simulink model "ieee14_fault"  (R2025b)
settings: Solver=ode23t  StartTime=0.0  StopTime=0.12  FixedStep=0.2  RelTol=1e-4  AbsTol=1e-6  EnableMultiTasking=on
undefined symbols (not defined in the file or in its folder): D1, Delta
libraries: spsDiodeLib x84, spsGroundLib x84, spsSeriesRLCBranchLib x84, spsDCVoltageSourceLib x84, spsBreakerLib x42, spsThreePhaseSeriesRLCBranchLib x20, spsThreePhaseVIMeasurementLib x16, spsThreePhaseFaultLib x14, spsThreePhaseSeriesRLCLoadLib x11, spsThreePhaseSourceLib x5, spsThreePhaseTransformerTwoWindingsLib x5, spspowerguiLib x1
(part 2 of 3)

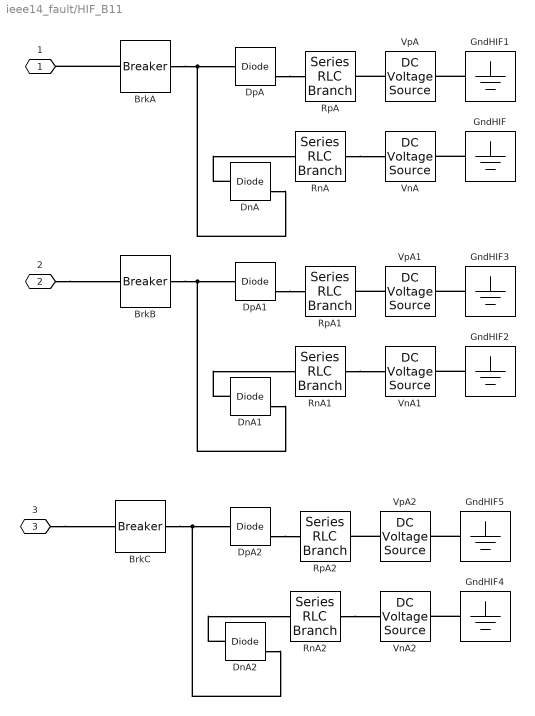
== system ieee14_fault/HIF_B11 ==
  BrkA : spsBreakerLib/Breaker  InitialState=0  SwitchingTimes=[100]  External=off  BreakerResistance=0.01  SnubberResistance=1e6  SnubberCapacitance=inf  Measurements=None  MoreParameters=on  NoBreakLoop=off
  BrkB : spsBreakerLib/Breaker  InitialState=0  SwitchingTimes=[100]  External=off  BreakerResistance=0.01  SnubberResistance=1e6  SnubberCapacitance=inf  Measurements=None  MoreParameters=on  NoBreakLoop=off
  BrkC : spsBreakerLib/Breaker  InitialState=0  SwitchingTimes=[100]  External=off  BreakerResistance=0.01  SnubberResistance=1e6  SnubberCapacitance=inf  Measurements=None  MoreParameters=on  NoBreakLoop=off
  DnA : spsDiodeLib/Diode  Ron=0.001  Lon=0  Vf=0.8  IC=0  UseSnubber=0  Rs=1e6  Cs=inf  Measurements=on
  DnA1 : spsDiodeLib/Diode  Ron=0.001  Lon=0  Vf=0.8  IC=0  UseSnubber=0  Rs=1e6  Cs=inf  Measurements=on
  DnA2 : spsDiodeLib/Diode  Ron=0.001  Lon=0  Vf=0.8  IC=0  UseSnubber=0  Rs=1e6  Cs=inf  Measurements=on
  DpA : spsDiodeLib/Diode  Ron=0.001  Lon=0  Vf=0.8  IC=0  UseSnubber=0  Rs=1e6  Cs=inf  Measurements=on
  DpA1 : spsDiodeLib/Diode  Ron=0.001  Lon=0  Vf=0.8  IC=0  UseSnubber=0  Rs=1e6  Cs=inf  Measurements=on
  DpA2 : spsDiodeLib/Diode  Ron=0.001  Lon=0  Vf=0.8  IC=0  UseSnubber=0  Rs=1e6  Cs=inf  Measurements=on
  GndHIF{,1..5} (6 alike) : spsGroundLib/Ground  LConnTagsString=a
  RnA : spsSeriesRLCBranchLib/Series RLC Branch  LConnTagsString=__new0  RConnTagsString=__new0  BranchType=R  Resistance=160  Inductance=1e-3  SetiL0=off  InitialCurrent=0  Capacitance=1e-6  Setx0=off  InitialVoltage=0  Measurements=None
  RnA1 : spsSeriesRLCBranchLib/Series RLC Branch  LConnTagsString=__new0  RConnTagsString=__new0  BranchType=R  Resistance=160  Inductance=1e-3  SetiL0=off  InitialCurrent=0  Capacitance=1e-6  Setx0=off  InitialVoltage=0  Measurements=None
  RnA2 : spsSeriesRLCBranchLib/Series RLC Branch  LConnTagsString=__new0  RConnTagsString=__new0  BranchType=R  Resistance=160  Inductance=1e-3  SetiL0=off  InitialCurrent=0  Capacitance=1e-6  Setx0=off  InitialVoltage=0  Measurements=None
  RpA : spsSeriesRLCBranchLib/Series RLC Branch  LConnTagsString=__new0  RConnTagsString=__new0  BranchType=R  Resistance=150  Inductance=1e-3  SetiL0=off  InitialCurrent=0  Capacitance=1e-6  Setx0=off  InitialVoltage=0  Measurements=None
  RpA1 : spsSeriesRLCBranchLib/Series RLC Branch  LConnTagsString=__new0  RConnTagsString=__new0  BranchType=R  Resistance=150  Inductance=1e-3  SetiL0=off  InitialCurrent=0  Capacitance=1e-6  Setx0=off  InitialVoltage=0  Measurements=None
  RpA2 : spsSeriesRLCBranchLib/Series RLC Branch  LConnTagsString=__new0  RConnTagsString=__new0  BranchType=R  Resistance=150  Inductance=1e-3  SetiL0=off  InitialCurrent=0  Capacitance=1e-6  Setx0=off  InitialVoltage=0  Measurements=None
  VnA : spsDCVoltageSourceLib/DC Voltage Source  Amplitude=2050  Measurements=None
  VnA1 : spsDCVoltageSourceLib/DC Voltage Source  Amplitude=2050  Measurements=None
  VnA2 : spsDCVoltageSourceLib/DC Voltage Source  Amplitude=2050  Measurements=None
  VpA : spsDCVoltageSourceLib/DC Voltage Source  Amplitude=2000  Measurements=None
  VpA1 : spsDCVoltageSourceLib/DC Voltage Source  Amplitude=2000  Measurements=None
  VpA2 : spsDCVoltageSourceLib/DC Voltage Source  Amplitude=2000  Measurements=None
  1 : PMIOPort  Side=Left
  2 : PMIOPort  Port=2  Side=Left
  3 : PMIOPort  Port=3  Side=Left
  connections:
  GndHIF3/LConn1 -- VpA1/LConn1
  DnA1/RConn1 -- DpA1/LConn1 -- BrkB/RConn1
  GndHIF5/LConn1 -- VpA2/LConn1
  VpA/RConn1 -- RpA/RConn1
  BrkA/LConn1 -- 1/RConn1
  DnA/LConn1 -- RnA/LConn1
  RnA1/RConn1 -- VnA1/LConn1
  DnA2/RConn1 -- DpA2/LConn1 -- BrkC/RConn1
  RnA2/RConn1 -- VnA2/LConn1
  VpA1/RConn1 -- RpA1/RConn1
  GndHIF2/LConn1 -- VnA1/RConn1
  DnA1/LConn1 -- RnA1/LConn1
  DpA2/RConn1 -- RpA2/LConn1
  GndHIF4/LConn1 -- VnA2/RConn1
  RnA/RConn1 -- VnA/LConn1
  VpA2/RConn1 -- RpA2/RConn1
  DnA2/LConn1 -- RnA2/LConn1
  DpA1/RConn1 -- RpA1/LConn1
  BrkA/RConn1 -- DpA/LConn1 -- DnA/RConn1
  GndHIF1/LConn1 -- VpA/LConn1
  DpA/RConn1 -- RpA/LConn1
  GndHIF/LConn1 -- VnA/RConn1
  2/RConn1 -- BrkB/LConn1
  3/RConn1 -- BrkC/LConn1

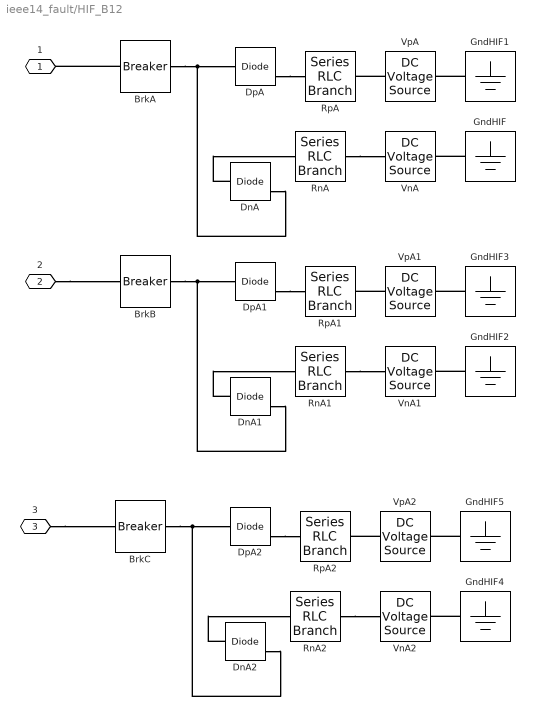
== system ieee14_fault/HIF_B12 ==
  BrkA : spsBreakerLib/Breaker  InitialState=0  SwitchingTimes=[100]  External=off  BreakerResistance=0.01  SnubberResistance=1e6  SnubberCapacitance=inf  Measurements=None  MoreParameters=on  NoBreakLoop=off
  BrkB : spsBreakerLib/Breaker  InitialState=0  SwitchingTimes=[100]  External=off  BreakerResistance=0.01  SnubberResistance=1e6  SnubberCapacitance=inf  Measurements=None  MoreParameters=on  NoBreakLoop=off
  BrkC : spsBreakerLib/Breaker  InitialState=0  SwitchingTimes=[100]  External=off  BreakerResistance=0.01  SnubberResistance=1e6  SnubberCapacitance=inf  Measurements=None  MoreParameters=on  NoBreakLoop=off
  DnA : spsDiodeLib/Diode  Ron=0.001  Lon=0  Vf=0.8  IC=0  UseSnubber=0  Rs=1e6  Cs=inf  Measurements=on
  DnA1 : spsDiodeLib/Diode  Ron=0.001  Lon=0  Vf=0.8  IC=0  UseSnubber=0  Rs=1e6  Cs=inf  Measurements=on
  DnA2 : spsDiodeLib/Diode  Ron=0.001  Lon=0  Vf=0.8  IC=0  UseSnubber=0  Rs=1e6  Cs=inf  Measurements=on
  DpA : spsDiodeLib/Diode  Ron=0.001  Lon=0  Vf=0.8  IC=0  UseSnubber=0  Rs=1e6  Cs=inf  Measurements=on
  DpA1 : spsDiodeLib/Diode  Ron=0.001  Lon=0  Vf=0.8  IC=0  UseSnubber=0  Rs=1e6  Cs=inf  Measurements=on
  DpA2 : spsDiodeLib/Diode  Ron=0.001  Lon=0  Vf=0.8  IC=0  UseSnubber=0  Rs=1e6  Cs=inf  Measurements=on
  GndHIF{,1..5} (6 alike) : spsGroundLib/Ground  LConnTagsString=a
  RnA : spsSeriesRLCBranchLib/Series RLC Branch  LConnTagsString=__new0  RConnTagsString=__new0  BranchType=R  Resistance=160  Inductance=1e-3  SetiL0=off  InitialCurrent=0  Capacitance=1e-6  Setx0=off  InitialVoltage=0  Measurements=None
  RnA1 : spsSeriesRLCBranchLib/Series RLC Branch  LConnTagsString=__new0  RConnTagsString=__new0  BranchType=R  Resistance=160  Inductance=1e-3  SetiL0=off  InitialCurrent=0  Capacitance=1e-6  Setx0=off  InitialVoltage=0  Measurements=None
  RnA2 : spsSeriesRLCBranchLib/Series RLC Branch  LConnTagsString=__new0  RConnTagsString=__new0  BranchType=R  Resistance=160  Inductance=1e-3  SetiL0=off  InitialCurrent=0  Capacitance=1e-6  Setx0=off  InitialVoltage=0  Measurements=None
  RpA : spsSeriesRLCBranchLib/Series RLC Branch  LConnTagsString=__new0  RConnTagsString=__new0  BranchType=R  Resistance=150  Inductance=1e-3  SetiL0=off  InitialCurrent=0  Capacitance=1e-6  Setx0=off  InitialVoltage=0  Measurements=None
  RpA1 : spsSeriesRLCBranchLib/Series RLC Branch  LConnTagsString=__new0  RConnTagsString=__new0  BranchType=R  Resistance=150  Inductance=1e-3  SetiL0=off  InitialCurrent=0  Capacitance=1e-6  Setx0=off  InitialVoltage=0  Measurements=None
  RpA2 : spsSeriesRLCBranchLib/Series RLC Branch  LConnTagsString=__new0  RConnTagsString=__new0  BranchType=R  Resistance=150  Inductance=1e-3  SetiL0=off  InitialCurrent=0  Capacitance=1e-6  Setx0=off  InitialVoltage=0  Measurements=None
  VnA : spsDCVoltageSourceLib/DC Voltage Source  Amplitude=2050  Measurements=None
  VnA1 : spsDCVoltageSourceLib/DC Voltage Source  Amplitude=2050  Measurements=None
  VnA2 : spsDCVoltageSourceLib/DC Voltage Source  Amplitude=2050  Measurements=None
  VpA : spsDCVoltageSourceLib/DC Voltage Source  Amplitude=2000  Measurements=None
  VpA1 : spsDCVoltageSourceLib/DC Voltage Source  Amplitude=2000  Measurements=None
  VpA2 : spsDCVoltageSourceLib/DC Voltage Source  Amplitude=2000  Measurements=None
  1 : PMIOPort  Side=Left
  2 : PMIOPort  Port=2  Side=Left
  3 : PMIOPort  Port=3  Side=Left
  connections:
  GndHIF3/LConn1 -- VpA1/LConn1
  DnA1/RConn1 -- DpA1/LConn1 -- BrkB/RConn1
  GndHIF5/LConn1 -- VpA2/LConn1
  VpA/RConn1 -- RpA/RConn1
  BrkA/LConn1 -- 1/RConn1
  DnA/LConn1 -- RnA/LConn1
  RnA1/RConn1 -- VnA1/LConn1
  DnA2/RConn1 -- DpA2/LConn1 -- BrkC/RConn1
  RnA2/RConn1 -- VnA2/LConn1
  VpA1/RConn1 -- RpA1/RConn1
  GndHIF2/LConn1 -- VnA1/RConn1
  DnA1/LConn1 -- RnA1/LConn1
  DpA2/RConn1 -- RpA2/LConn1
  GndHIF4/LConn1 -- VnA2/RConn1
  RnA/RConn1 -- VnA/LConn1
  VpA2/RConn1 -- RpA2/RConn1
  DnA2/LConn1 -- RnA2/LConn1
  DpA1/RConn1 -- RpA1/LConn1
  BrkA/RConn1 -- DpA/LConn1 -- DnA/RConn1
  GndHIF1/LConn1 -- VpA/LConn1
  DpA/RConn1 -- RpA/LConn1
  GndHIF/LConn1 -- VnA/RConn1
  2/RConn1 -- BrkB/LConn1
  3/RConn1 -- BrkC/LConn1

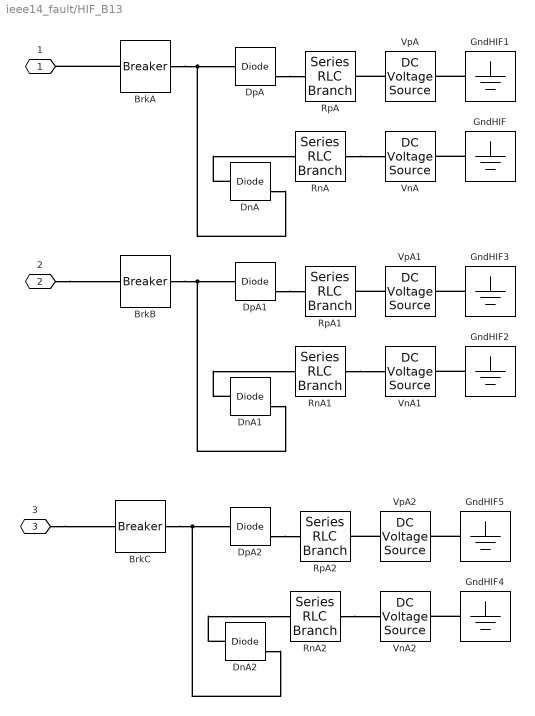
== system ieee14_fault/HIF_B13 ==
  BrkA : spsBreakerLib/Breaker  InitialState=0  SwitchingTimes=[100]  External=off  BreakerResistance=0.01  SnubberResistance=1e6  SnubberCapacitance=inf  Measurements=None  MoreParameters=on  NoBreakLoop=off
  BrkB : spsBreakerLib/Breaker  InitialState=0  SwitchingTimes=[100]  External=off  BreakerResistance=0.01  SnubberResistance=1e6  SnubberCapacitance=inf  Measurements=None  MoreParameters=on  NoBreakLoop=off
  BrkC : spsBreakerLib/Breaker  InitialState=0  SwitchingTimes=[100]  External=off  BreakerResistance=0.01  SnubberResistance=1e6  SnubberCapacitance=inf  Measurements=None  MoreParameters=on  NoBreakLoop=off
  DnA : spsDiodeLib/Diode  Ron=0.001  Lon=0  Vf=0.8  IC=0  UseSnubber=0  Rs=1e6  Cs=inf  Measurements=on
  DnA1 : spsDiodeLib/Diode  Ron=0.001  Lon=0  Vf=0.8  IC=0  UseSnubber=0  Rs=1e6  Cs=inf  Measurements=on
  DnA2 : spsDiodeLib/Diode  Ron=0.001  Lon=0  Vf=0.8  IC=0  UseSnubber=0  Rs=1e6  Cs=inf  Measurements=on
  DpA : spsDiodeLib/Diode  Ron=0.001  Lon=0  Vf=0.8  IC=0  UseSnubber=0  Rs=1e6  Cs=inf  Measurements=on
  DpA1 : spsDiodeLib/Diode  Ron=0.001  Lon=0  Vf=0.8  IC=0  UseSnubber=0  Rs=1e6  Cs=inf  Measurements=on
  DpA2 : spsDiodeLib/Diode  Ron=0.001  Lon=0  Vf=0.8  IC=0  UseSnubber=0  Rs=1e6  Cs=inf  Measurements=on
  GndHIF{,1..5} (6 alike) : spsGroundLib/Ground  LConnTagsString=a
  RnA : spsSeriesRLCBranchLib/Series RLC Branch  LConnTagsString=__new0  RConnTagsString=__new0  BranchType=R  Resistance=160  Inductance=1e-3  SetiL0=off  InitialCurrent=0  Capacitance=1e-6  Setx0=off  InitialVoltage=0  Measurements=None
  RnA1 : spsSeriesRLCBranchLib/Series RLC Branch  LConnTagsString=__new0  RConnTagsString=__new0  BranchType=R  Resistance=160  Inductance=1e-3  SetiL0=off  InitialCurrent=0  Capacitance=1e-6  Setx0=off  InitialVoltage=0  Measurements=None
  RnA2 : spsSeriesRLCBranchLib/Series RLC Branch  LConnTagsString=__new0  RConnTagsString=__new0  BranchType=R  Resistance=160  Inductance=1e-3  SetiL0=off  InitialCurrent=0  Capacitance=1e-6  Setx0=off  InitialVoltage=0  Measurements=None
  RpA : spsSeriesRLCBranchLib/Series RLC Branch  LConnTagsString=__new0  RConnTagsString=__new0  BranchType=R  Resistance=150  Inductance=1e-3  SetiL0=off  InitialCurrent=0  Capacitance=1e-6  Setx0=off  InitialVoltage=0  Measurements=None
  RpA1 : spsSeriesRLCBranchLib/Series RLC Branch  LConnTagsString=__new0  RConnTagsString=__new0  BranchType=R  Resistance=150  Inductance=1e-3  SetiL0=off  InitialCurrent=0  Capacitance=1e-6  Setx0=off  InitialVoltage=0  Measurements=None
  RpA2 : spsSeriesRLCBranchLib/Series RLC Branch  LConnTagsString=__new0  RConnTagsString=__new0  BranchType=R  Resistance=150  Inductance=1e-3  SetiL0=off  InitialCurrent=0  Capacitance=1e-6  Setx0=off  InitialVoltage=0  Measurements=None
  VnA : spsDCVoltageSourceLib/DC Voltage Source  Amplitude=2050  Measurements=None
  VnA1 : spsDCVoltageSourceLib/DC Voltage Source  Amplitude=2050  Measurements=None
  VnA2 : spsDCVoltageSourceLib/DC Voltage Source  Amplitude=2050  Measurements=None
  VpA : spsDCVoltageSourceLib/DC Voltage Source  Amplitude=2000  Measurements=None
  VpA1 : spsDCVoltageSourceLib/DC Voltage Source  Amplitude=2000  Measurements=None
  VpA2 : spsDCVoltageSourceLib/DC Voltage Source  Amplitude=2000  Measurements=None
  1 : PMIOPort  Side=Left
  2 : PMIOPort  Port=2  Side=Left
  3 : PMIOPort  Port=3  Side=Left
  connections:
  GndHIF3/LConn1 -- VpA1/LConn1
  DnA1/RConn1 -- DpA1/LConn1 -- BrkB/RConn1
  GndHIF5/LConn1 -- VpA2/LConn1
  VpA/RConn1 -- RpA/RConn1
  BrkA/LConn1 -- 1/RConn1
  DnA/LConn1 -- RnA/LConn1
  RnA1/RConn1 -- VnA1/LConn1
  DnA2/RConn1 -- DpA2/LConn1 -- BrkC/RConn1
  RnA2/RConn1 -- VnA2/LConn1
  VpA1/RConn1 -- RpA1/RConn1
  GndHIF2/LConn1 -- VnA1/RConn1
  DnA1/LConn1 -- RnA1/LConn1
  DpA2/RConn1 -- RpA2/LConn1
  GndHIF4/LConn1 -- VnA2/RConn1
  RnA/RConn1 -- VnA/LConn1
  VpA2/RConn1 -- RpA2/RConn1
  DnA2/LConn1 -- RnA2/LConn1
  DpA1/RConn1 -- RpA1/LConn1
  BrkA/RConn1 -- DpA/LConn1 -- DnA/RConn1
  GndHIF1/LConn1 -- VpA/LConn1
  DpA/RConn1 -- RpA/LConn1
  GndHIF/LConn1 -- VnA/RConn1
  2/RConn1 -- BrkB/LConn1
  3/RConn1 -- BrkC/LConn1

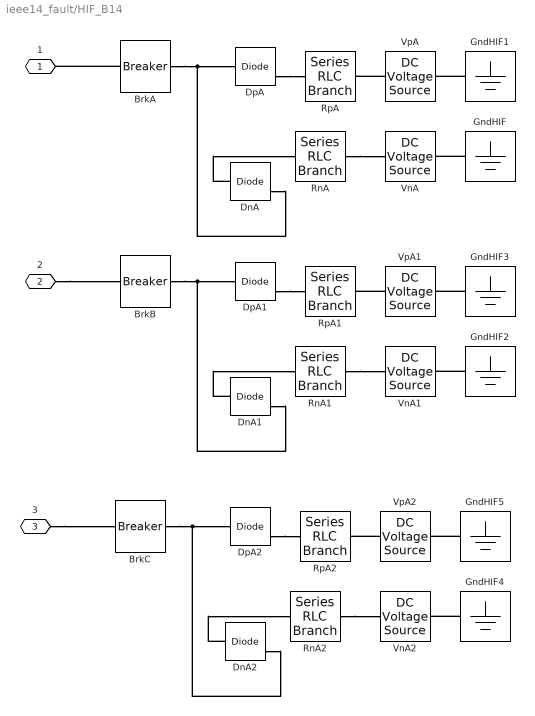
== system ieee14_fault/HIF_B14 ==
  BrkA : spsBreakerLib/Breaker  InitialState=0  SwitchingTimes=[100]  External=off  BreakerResistance=0.01  SnubberResistance=1e6  SnubberCapacitance=inf  Measurements=None  MoreParameters=on  NoBreakLoop=off
  BrkB : spsBreakerLib/Breaker  InitialState=0  SwitchingTimes=[100]  External=off  BreakerResistance=0.01  SnubberResistance=1e6  SnubberCapacitance=inf  Measurements=None  MoreParameters=on  NoBreakLoop=off
  BrkC : spsBreakerLib/Breaker  InitialState=0  SwitchingTimes=[100]  External=off  BreakerResistance=0.01  SnubberResistance=1e6  SnubberCapacitance=inf  Measurements=None  MoreParameters=on  NoBreakLoop=off
  DnA : spsDiodeLib/Diode  Ron=0.001  Lon=0  Vf=0.8  IC=0  UseSnubber=0  Rs=1e6  Cs=inf  Measurements=on
  DnA1 : spsDiodeLib/Diode  Ron=0.001  Lon=0  Vf=0.8  IC=0  UseSnubber=0  Rs=1e6  Cs=inf  Measurements=on
  DnA2 : spsDiodeLib/Diode  Ron=0.001  Lon=0  Vf=0.8  IC=0  UseSnubber=0  Rs=1e6  Cs=inf  Measurements=on
  DpA : spsDiodeLib/Diode  Ron=0.001  Lon=0  Vf=0.8  IC=0  UseSnubber=0  Rs=1e6  Cs=inf  Measurements=on
  DpA1 : spsDiodeLib/Diode  Ron=0.001  Lon=0  Vf=0.8  IC=0  UseSnubber=0  Rs=1e6  Cs=inf  Measurements=on
  DpA2 : spsDiodeLib/Diode  Ron=0.001  Lon=0  Vf=0.8  IC=0  UseSnubber=0  Rs=1e6  Cs=inf  Measurements=on
  GndHIF{,1..5} (6 alike) : spsGroundLib/Ground  LConnTagsString=a
  RnA : spsSeriesRLCBranchLib/Series RLC Branch  LConnTagsString=__new0  RConnTagsString=__new0  BranchType=R  Resistance=160  Inductance=1e-3  SetiL0=off  InitialCurrent=0  Capacitance=1e-6  Setx0=off  InitialVoltage=0  Measurements=None
  RnA1 : spsSeriesRLCBranchLib/Series RLC Branch  LConnTagsString=__new0  RConnTagsString=__new0  BranchType=R  Resistance=160  Inductance=1e-3  SetiL0=off  InitialCurrent=0  Capacitance=1e-6  Setx0=off  InitialVoltage=0  Measurements=None
  RnA2 : spsSeriesRLCBranchLib/Series RLC Branch  LConnTagsString=__new0  RConnTagsString=__new0  BranchType=R  Resistance=160  Inductance=1e-3  SetiL0=off  InitialCurrent=0  Capacitance=1e-6  Setx0=off  InitialVoltage=0  Measurements=None
  RpA : spsSeriesRLCBranchLib/Series RLC Branch  LConnTagsString=__new0  RConnTagsString=__new0  BranchType=R  Resistance=150  Inductance=1e-3  SetiL0=off  InitialCurrent=0  Capacitance=1e-6  Setx0=off  InitialVoltage=0  Measurements=None
  RpA1 : spsSeriesRLCBranchLib/Series RLC Branch  LConnTagsString=__new0  RConnTagsString=__new0  BranchType=R  Resistance=150  Inductance=1e-3  SetiL0=off  InitialCurrent=0  Capacitance=1e-6  Setx0=off  InitialVoltage=0  Measurements=None
  RpA2 : spsSeriesRLCBranchLib/Series RLC Branch  LConnTagsString=__new0  RConnTagsString=__new0  BranchType=R  Resistance=150  Inductance=1e-3  SetiL0=off  InitialCurrent=0  Capacitance=1e-6  Setx0=off  InitialVoltage=0  Measurements=None
  VnA : spsDCVoltageSourceLib/DC Voltage Source  Amplitude=2050  Measurements=None
  VnA1 : spsDCVoltageSourceLib/DC Voltage Source  Amplitude=2050  Measurements=None
  VnA2 : spsDCVoltageSourceLib/DC Voltage Source  Amplitude=2050  Measurements=None
  VpA : spsDCVoltageSourceLib/DC Voltage Source  Amplitude=2000  Measurements=None
  VpA1 : spsDCVoltageSourceLib/DC Voltage Source  Amplitude=2000  Measurements=None
  VpA2 : spsDCVoltageSourceLib/DC Voltage Source  Amplitude=2000  Measurements=None
  1 : PMIOPort  Side=Left
  2 : PMIOPort  Port=2  Side=Left
  3 : PMIOPort  Port=3  Side=Left
  connections:
  GndHIF3/LConn1 -- VpA1/LConn1
  DnA1/RConn1 -- DpA1/LConn1 -- BrkB/RConn1
  GndHIF5/LConn1 -- VpA2/LConn1
  VpA/RConn1 -- RpA/RConn1
  BrkA/LConn1 -- 1/RConn1
  DnA/LConn1 -- RnA/LConn1
  RnA1/RConn1 -- VnA1/LConn1
  DnA2/RConn1 -- DpA2/LConn1 -- BrkC/RConn1
  RnA2/RConn1 -- VnA2/LConn1
  VpA1/RConn1 -- RpA1/RConn1
  GndHIF2/LConn1 -- VnA1/RConn1
  DnA1/LConn1 -- RnA1/LConn1
  DpA2/RConn1 -- RpA2/LConn1
  GndHIF4/LConn1 -- VnA2/RConn1
  RnA/RConn1 -- VnA/LConn1
  VpA2/RConn1 -- RpA2/RConn1
  DnA2/LConn1 -- RnA2/LConn1
  DpA1/RConn1 -- RpA1/LConn1
  BrkA/RConn1 -- DpA/LConn1 -- DnA/RConn1
  GndHIF1/LConn1 -- VpA/LConn1
  DpA/RConn1 -- RpA/LConn1
  GndHIF/LConn1 -- VnA/RConn1
  2/RConn1 -- BrkB/LConn1
  3/RConn1 -- BrkC/LConn1

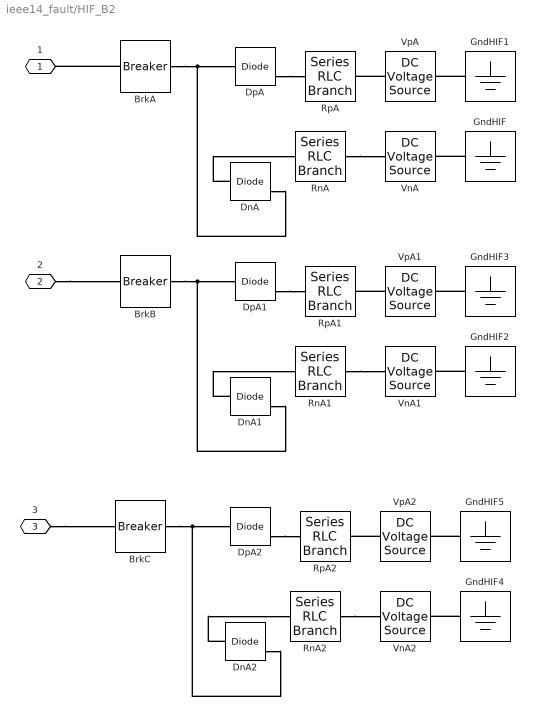
== system ieee14_fault/HIF_B2 ==
  BrkA : spsBreakerLib/Breaker  InitialState=0  SwitchingTimes=[100]  External=off  BreakerResistance=0.01  SnubberResistance=1e6  SnubberCapacitance=inf  Measurements=None  MoreParameters=on  NoBreakLoop=off
  BrkB : spsBreakerLib/Breaker  InitialState=0  SwitchingTimes=[100]  External=off  BreakerResistance=0.01  SnubberResistance=1e6  SnubberCapacitance=inf  Measurements=None  MoreParameters=on  NoBreakLoop=off
  BrkC : spsBreakerLib/Breaker  InitialState=0  SwitchingTimes=[100]  External=off  BreakerResistance=0.01  SnubberResistance=1e6  SnubberCapacitance=inf  Measurements=None  MoreParameters=on  NoBreakLoop=off
  DnA : spsDiodeLib/Diode  Ron=0.001  Lon=0  Vf=0.8  IC=0  UseSnubber=0  Rs=1e6  Cs=inf  Measurements=on
  DnA1 : spsDiodeLib/Diode  Ron=0.001  Lon=0  Vf=0.8  IC=0  UseSnubber=0  Rs=1e6  Cs=inf  Measurements=on
  DnA2 : spsDiodeLib/Diode  Ron=0.001  Lon=0  Vf=0.8  IC=0  UseSnubber=0  Rs=1e6  Cs=inf  Measurements=on
  DpA : spsDiodeLib/Diode  Ron=0.001  Lon=0  Vf=0.8  IC=0  UseSnubber=0  Rs=1e6  Cs=inf  Measurements=on
  DpA1 : spsDiodeLib/Diode  Ron=0.001  Lon=0  Vf=0.8  IC=0  UseSnubber=0  Rs=1e6  Cs=inf  Measurements=on
  DpA2 : spsDiodeLib/Diode  Ron=0.001  Lon=0  Vf=0.8  IC=0  UseSnubber=0  Rs=1e6  Cs=inf  Measurements=on
  GndHIF{,1..5} (6 alike) : spsGroundLib/Ground  LConnTagsString=a
  RnA : spsSeriesRLCBranchLib/Series RLC Branch  LConnTagsString=__new0  RConnTagsString=__new0  BranchType=R  Resistance=160  Inductance=1e-3  SetiL0=off  InitialCurrent=0  Capacitance=1e-6  Setx0=off  InitialVoltage=0  Measurements=None
  RnA1 : spsSeriesRLCBranchLib/Series RLC Branch  LConnTagsString=__new0  RConnTagsString=__new0  BranchType=R  Resistance=160  Inductance=1e-3  SetiL0=off  InitialCurrent=0  Capacitance=1e-6  Setx0=off  InitialVoltage=0  Measurements=None
  RnA2 : spsSeriesRLCBranchLib/Series RLC Branch  LConnTagsString=__new0  RConnTagsString=__new0  BranchType=R  Resistance=160  Inductance=1e-3  SetiL0=off  InitialCurrent=0  Capacitance=1e-6  Setx0=off  InitialVoltage=0  Measurements=None
  RpA : spsSeriesRLCBranchLib/Series RLC Branch  LConnTagsString=__new0  RConnTagsString=__new0  BranchType=R  Resistance=150  Inductance=1e-3  SetiL0=off  InitialCurrent=0  Capacitance=1e-6  Setx0=off  InitialVoltage=0  Measurements=None
  RpA1 : spsSeriesRLCBranchLib/Series RLC Branch  LConnTagsString=__new0  RConnTagsString=__new0  BranchType=R  Resistance=150  Inductance=1e-3  SetiL0=off  InitialCurrent=0  Capacitance=1e-6  Setx0=off  InitialVoltage=0  Measurements=None
  RpA2 : spsSeriesRLCBranchLib/Series RLC Branch  LConnTagsString=__new0  RConnTagsString=__new0  BranchType=R  Resistance=150  Inductance=1e-3  SetiL0=off  InitialCurrent=0  Capacitance=1e-6  Setx0=off  InitialVoltage=0  Measurements=None
  VnA : spsDCVoltageSourceLib/DC Voltage Source  Amplitude=2050  Measurements=None
  VnA1 : spsDCVoltageSourceLib/DC Voltage Source  Amplitude=2050  Measurements=None
  VnA2 : spsDCVoltageSourceLib/DC Voltage Source  Amplitude=2050  Measurements=None
  VpA : spsDCVoltageSourceLib/DC Voltage Source  Amplitude=2000  Measurements=None
  VpA1 : spsDCVoltageSourceLib/DC Voltage Source  Amplitude=2000  Measurements=None
  VpA2 : spsDCVoltageSourceLib/DC Voltage Source  Amplitude=2000  Measurements=None
  1 : PMIOPort  Side=Left
  2 : PMIOPort  Port=2  Side=Left
  3 : PMIOPort  Port=3  Side=Left
  connections:
  GndHIF3/LConn1 -- VpA1/LConn1
  DnA1/RConn1 -- DpA1/LConn1 -- BrkB/RConn1
  GndHIF5/LConn1 -- VpA2/LConn1
  VpA/RConn1 -- RpA/RConn1
  BrkA/LConn1 -- 1/RConn1
  DnA/LConn1 -- RnA/LConn1
  RnA1/RConn1 -- VnA1/LConn1
  DnA2/RConn1 -- DpA2/LConn1 -- BrkC/RConn1
  RnA2/RConn1 -- VnA2/LConn1
  VpA1/RConn1 -- RpA1/RConn1
  GndHIF2/LConn1 -- VnA1/RConn1
  DnA1/LConn1 -- RnA1/LConn1
  DpA2/RConn1 -- RpA2/LConn1
  GndHIF4/LConn1 -- VnA2/RConn1
  RnA/RConn1 -- VnA/LConn1
  VpA2/RConn1 -- RpA2/RConn1
  DnA2/LConn1 -- RnA2/LConn1
  DpA1/RConn1 -- RpA1/LConn1
  BrkA/RConn1 -- DpA/LConn1 -- DnA/RConn1
  GndHIF1/LConn1 -- VpA/LConn1
  DpA/RConn1 -- RpA/LConn1
  GndHIF/LConn1 -- VnA/RConn1
  2/RConn1 -- BrkB/LConn1
  3/RConn1 -- BrkC/LConn1

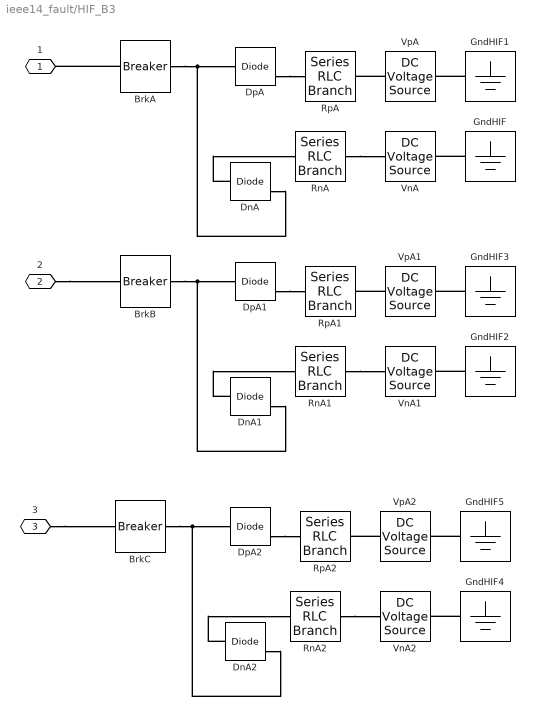
== system ieee14_fault/HIF_B3 ==
  BrkA : spsBreakerLib/Breaker  InitialState=0  SwitchingTimes=[100]  External=off  BreakerResistance=0.01  SnubberResistance=1e6  SnubberCapacitance=inf  Measurements=None  MoreParameters=on  NoBreakLoop=off
  BrkB : spsBreakerLib/Breaker  InitialState=0  SwitchingTimes=[100]  External=off  BreakerResistance=0.01  SnubberResistance=1e6  SnubberCapacitance=inf  Measurements=None  MoreParameters=on  NoBreakLoop=off
  BrkC : spsBreakerLib/Breaker  InitialState=0  SwitchingTimes=[100]  External=off  BreakerResistance=0.01  SnubberResistance=1e6  SnubberCapacitance=inf  Measurements=None  MoreParameters=on  NoBreakLoop=off
  DnA : spsDiodeLib/Diode  Ron=0.001  Lon=0  Vf=0.8  IC=0  UseSnubber=0  Rs=1e6  Cs=inf  Measurements=on
  DnA1 : spsDiodeLib/Diode  Ron=0.001  Lon=0  Vf=0.8  IC=0  UseSnubber=0  Rs=1e6  Cs=inf  Measurements=on
  DnA2 : spsDiodeLib/Diode  Ron=0.001  Lon=0  Vf=0.8  IC=0  UseSnubber=0  Rs=1e6  Cs=inf  Measurements=on
  DpA : spsDiodeLib/Diode  Ron=0.001  Lon=0  Vf=0.8  IC=0  UseSnubber=0  Rs=1e6  Cs=inf  Measurements=on
  DpA1 : spsDiodeLib/Diode  Ron=0.001  Lon=0  Vf=0.8  IC=0  UseSnubber=0  Rs=1e6  Cs=inf  Measurements=on
  DpA2 : spsDiodeLib/Diode  Ron=0.001  Lon=0  Vf=0.8  IC=0  UseSnubber=0  Rs=1e6  Cs=inf  Measurements=on
  GndHIF{,1..5} (6 alike) : spsGroundLib/Ground  LConnTagsString=a
  RnA : spsSeriesRLCBranchLib/Series RLC Branch  LConnTagsString=__new0  RConnTagsString=__new0  BranchType=R  Resistance=160  Inductance=1e-3  SetiL0=off  InitialCurrent=0  Capacitance=1e-6  Setx0=off  InitialVoltage=0  Measurements=None
  RnA1 : spsSeriesRLCBranchLib/Series RLC Branch  LConnTagsString=__new0  RConnTagsString=__new0  BranchType=R  Resistance=160  Inductance=1e-3  SetiL0=off  InitialCurrent=0  Capacitance=1e-6  Setx0=off  InitialVoltage=0  Measurements=None
  RnA2 : spsSeriesRLCBranchLib/Series RLC Branch  LConnTagsString=__new0  RConnTagsString=__new0  BranchType=R  Resistance=160  Inductance=1e-3  SetiL0=off  InitialCurrent=0  Capacitance=1e-6  Setx0=off  InitialVoltage=0  Measurements=None
  RpA : spsSeriesRLCBranchLib/Series RLC Branch  LConnTagsString=__new0  RConnTagsString=__new0  BranchType=R  Resistance=150  Inductance=1e-3  SetiL0=off  InitialCurrent=0  Capacitance=1e-6  Setx0=off  InitialVoltage=0  Measurements=None
  RpA1 : spsSeriesRLCBranchLib/Series RLC Branch  LConnTagsString=__new0  RConnTagsString=__new0  BranchType=R  Resistance=150  Inductance=1e-3  SetiL0=off  InitialCurrent=0  Capacitance=1e-6  Setx0=off  InitialVoltage=0  Measurements=None
  RpA2 : spsSeriesRLCBranchLib/Series RLC Branch  LConnTagsString=__new0  RConnTagsString=__new0  BranchType=R  Resistance=150  Inductance=1e-3  SetiL0=off  InitialCurrent=0  Capacitance=1e-6  Setx0=off  InitialVoltage=0  Measurements=None
  VnA : spsDCVoltageSourceLib/DC Voltage Source  Amplitude=2050  Measurements=None
  VnA1 : spsDCVoltageSourceLib/DC Voltage Source  Amplitude=2050  Measurements=None
  VnA2 : spsDCVoltageSourceLib/DC Voltage Source  Amplitude=2050  Measurements=None
  VpA : spsDCVoltageSourceLib/DC Voltage Source  Amplitude=2000  Measurements=None
  VpA1 : spsDCVoltageSourceLib/DC Voltage Source  Amplitude=2000  Measurements=None
  VpA2 : spsDCVoltageSourceLib/DC Voltage Source  Amplitude=2000  Measurements=None
  1 : PMIOPort  Side=Left
  2 : PMIOPort  Port=2  Side=Left
  3 : PMIOPort  Port=3  Side=Left
  connections:
  GndHIF3/LConn1 -- VpA1/LConn1
  DnA1/RConn1 -- DpA1/LConn1 -- BrkB/RConn1
  GndHIF5/LConn1 -- VpA2/LConn1
  VpA/RConn1 -- RpA/RConn1
  BrkA/LConn1 -- 1/RConn1
  DnA/LConn1 -- RnA/LConn1
  RnA1/RConn1 -- VnA1/LConn1
  DnA2/RConn1 -- DpA2/LConn1 -- BrkC/RConn1
  RnA2/RConn1 -- VnA2/LConn1
  VpA1/RConn1 -- RpA1/RConn1
  GndHIF2/LConn1 -- VnA1/RConn1
  DnA1/LConn1 -- RnA1/LConn1
  DpA2/RConn1 -- RpA2/LConn1
  GndHIF4/LConn1 -- VnA2/RConn1
  RnA/RConn1 -- VnA/LConn1
  VpA2/RConn1 -- RpA2/RConn1
  DnA2/LConn1 -- RnA2/LConn1
  DpA1/RConn1 -- RpA1/LConn1
  BrkA/RConn1 -- DpA/LConn1 -- DnA/RConn1
  GndHIF1/LConn1 -- VpA/LConn1
  DpA/RConn1 -- RpA/LConn1
  GndHIF/LConn1 -- VnA/RConn1
  2/RConn1 -- BrkB/LConn1
  3/RConn1 -- BrkC/LConn1

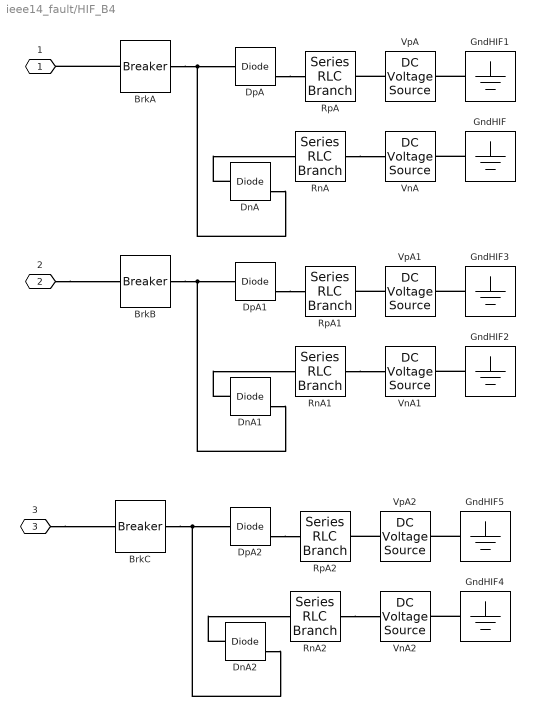
== system ieee14_fault/HIF_B4 ==
  BrkA : spsBreakerLib/Breaker  InitialState=0  SwitchingTimes=[100]  External=off  BreakerResistance=0.01  SnubberResistance=1e6  SnubberCapacitance=inf  Measurements=None  MoreParameters=on  NoBreakLoop=off
  BrkB : spsBreakerLib/Breaker  InitialState=0  SwitchingTimes=[100]  External=off  BreakerResistance=0.01  SnubberResistance=1e6  SnubberCapacitance=inf  Measurements=None  MoreParameters=on  NoBreakLoop=off
  BrkC : spsBreakerLib/Breaker  InitialState=0  SwitchingTimes=[100]  External=off  BreakerResistance=0.01  SnubberResistance=1e6  SnubberCapacitance=inf  Measurements=None  MoreParameters=on  NoBreakLoop=off
  DnA : spsDiodeLib/Diode  Ron=0.001  Lon=0  Vf=0.8  IC=0  UseSnubber=0  Rs=1e6  Cs=inf  Measurements=on
  DnA1 : spsDiodeLib/Diode  Ron=0.001  Lon=0  Vf=0.8  IC=0  UseSnubber=0  Rs=1e6  Cs=inf  Measurements=on
  DnA2 : spsDiodeLib/Diode  Ron=0.001  Lon=0  Vf=0.8  IC=0  UseSnubber=0  Rs=1e6  Cs=inf  Measurements=on
  DpA : spsDiodeLib/Diode  Ron=0.001  Lon=0  Vf=0.8  IC=0  UseSnubber=0  Rs=1e6  Cs=inf  Measurements=on
  DpA1 : spsDiodeLib/Diode  Ron=0.001  Lon=0  Vf=0.8  IC=0  UseSnubber=0  Rs=1e6  Cs=inf  Measurements=on
  DpA2 : spsDiodeLib/Diode  Ron=0.001  Lon=0  Vf=0.8  IC=0  UseSnubber=0  Rs=1e6  Cs=inf  Measurements=on
  GndHIF{,1..5} (6 alike) : spsGroundLib/Ground  LConnTagsString=a
  RnA : spsSeriesRLCBranchLib/Series RLC Branch  LConnTagsString=__new0  RConnTagsString=__new0  BranchType=R  Resistance=160  Inductance=1e-3  SetiL0=off  InitialCurrent=0  Capacitance=1e-6  Setx0=off  InitialVoltage=0  Measurements=None
  RnA1 : spsSeriesRLCBranchLib/Series RLC Branch  LConnTagsString=__new0  RConnTagsString=__new0  BranchType=R  Resistance=160  Inductance=1e-3  SetiL0=off  InitialCurrent=0  Capacitance=1e-6  Setx0=off  InitialVoltage=0  Measurements=None
  RnA2 : spsSeriesRLCBranchLib/Series RLC Branch  LConnTagsString=__new0  RConnTagsString=__new0  BranchType=R  Resistance=160  Inductance=1e-3  SetiL0=off  InitialCurrent=0  Capacitance=1e-6  Setx0=off  InitialVoltage=0  Measurements=None
  RpA : spsSeriesRLCBranchLib/Series RLC Branch  LConnTagsString=__new0  RConnTagsString=__new0  BranchType=R  Resistance=150  Inductance=1e-3  SetiL0=off  InitialCurrent=0  Capacitance=1e-6  Setx0=off  InitialVoltage=0  Measurements=None
  RpA1 : spsSeriesRLCBranchLib/Series RLC Branch  LConnTagsString=__new0  RConnTagsString=__new0  BranchType=R  Resistance=150  Inductance=1e-3  SetiL0=off  InitialCurrent=0  Capacitance=1e-6  Setx0=off  InitialVoltage=0  Measurements=None
  RpA2 : spsSeriesRLCBranchLib/Series RLC Branch  LConnTagsString=__new0  RConnTagsString=__new0  BranchType=R  Resistance=150  Inductance=1e-3  SetiL0=off  InitialCurrent=0  Capacitance=1e-6  Setx0=off  InitialVoltage=0  Measurements=None
  VnA : spsDCVoltageSourceLib/DC Voltage Source  Amplitude=2050  Measurements=None
  VnA1 : spsDCVoltageSourceLib/DC Voltage Source  Amplitude=2050  Measurements=None
  VnA2 : spsDCVoltageSourceLib/DC Voltage Source  Amplitude=2050  Measurements=None
  VpA : spsDCVoltageSourceLib/DC Voltage Source  Amplitude=2000  Measurements=None
  VpA1 : spsDCVoltageSourceLib/DC Voltage Source  Amplitude=2000  Measurements=None
  VpA2 : spsDCVoltageSourceLib/DC Voltage Source  Amplitude=2000  Measurements=None
  1 : PMIOPort  Side=Left
  2 : PMIOPort  Port=2  Side=Left
  3 : PMIOPort  Port=3  Side=Left
  connections:
  GndHIF3/LConn1 -- VpA1/LConn1
  DnA1/RConn1 -- DpA1/LConn1 -- BrkB/RConn1
  GndHIF5/LConn1 -- VpA2/LConn1
  VpA/RConn1 -- RpA/RConn1
  BrkA/LConn1 -- 1/RConn1
  DnA/LConn1 -- RnA/LConn1
  RnA1/RConn1 -- VnA1/LConn1
  DnA2/RConn1 -- DpA2/LConn1 -- BrkC/RConn1
  RnA2/RConn1 -- VnA2/LConn1
  VpA1/RConn1 -- RpA1/RConn1
  GndHIF2/LConn1 -- VnA1/RConn1
  DnA1/LConn1 -- RnA1/LConn1
  DpA2/RConn1 -- RpA2/LConn1
  GndHIF4/LConn1 -- VnA2/RConn1
  RnA/RConn1 -- VnA/LConn1
  VpA2/RConn1 -- RpA2/RConn1
  DnA2/LConn1 -- RnA2/LConn1
  DpA1/RConn1 -- RpA1/LConn1
  BrkA/RConn1 -- DpA/LConn1 -- DnA/RConn1
  GndHIF1/LConn1 -- VpA/LConn1
  DpA/RConn1 -- RpA/LConn1
  GndHIF/LConn1 -- VnA/RConn1
  2/RConn1 -- BrkB/LConn1
  3/RConn1 -- BrkC/LConn1

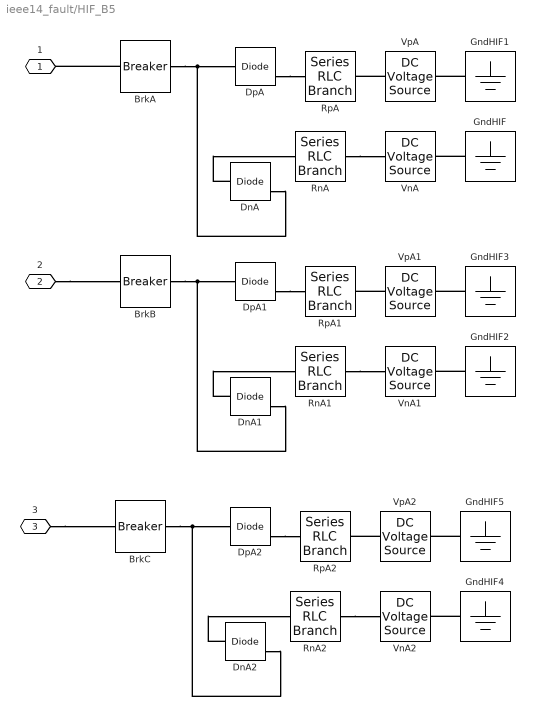
== system ieee14_fault/HIF_B5 ==
  BrkA : spsBreakerLib/Breaker  InitialState=0  SwitchingTimes=[100]  External=off  BreakerResistance=0.01  SnubberResistance=1e6  SnubberCapacitance=inf  Measurements=None  MoreParameters=on  NoBreakLoop=off
  BrkB : spsBreakerLib/Breaker  InitialState=0  SwitchingTimes=[100]  External=off  BreakerResistance=0.01  SnubberResistance=1e6  SnubberCapacitance=inf  Measurements=None  MoreParameters=on  NoBreakLoop=off
  BrkC : spsBreakerLib/Breaker  InitialState=0  SwitchingTimes=[100]  External=off  BreakerResistance=0.01  SnubberResistance=1e6  SnubberCapacitance=inf  Measurements=None  MoreParameters=on  NoBreakLoop=off
  DnA : spsDiodeLib/Diode  Ron=0.001  Lon=0  Vf=0.8  IC=0  UseSnubber=0  Rs=1e6  Cs=inf  Measurements=on
  DnA1 : spsDiodeLib/Diode  Ron=0.001  Lon=0  Vf=0.8  IC=0  UseSnubber=0  Rs=1e6  Cs=inf  Measurements=on
  DnA2 : spsDiodeLib/Diode  Ron=0.001  Lon=0  Vf=0.8  IC=0  UseSnubber=0  Rs=1e6  Cs=inf  Measurements=on
  DpA : spsDiodeLib/Diode  Ron=0.001  Lon=0  Vf=0.8  IC=0  UseSnubber=0  Rs=1e6  Cs=inf  Measurements=on
  DpA1 : spsDiodeLib/Diode  Ron=0.001  Lon=0  Vf=0.8  IC=0  UseSnubber=0  Rs=1e6  Cs=inf  Measurements=on
  DpA2 : spsDiodeLib/Diode  Ron=0.001  Lon=0  Vf=0.8  IC=0  UseSnubber=0  Rs=1e6  Cs=inf  Measurements=on
  GndHIF{,1..5} (6 alike) : spsGroundLib/Ground  LConnTagsString=a
  RnA : spsSeriesRLCBranchLib/Series RLC Branch  LConnTagsString=__new0  RConnTagsString=__new0  BranchType=R  Resistance=160  Inductance=1e-3  SetiL0=off  InitialCurrent=0  Capacitance=1e-6  Setx0=off  InitialVoltage=0  Measurements=None
  RnA1 : spsSeriesRLCBranchLib/Series RLC Branch  LConnTagsString=__new0  RConnTagsString=__new0  BranchType=R  Resistance=160  Inductance=1e-3  SetiL0=off  InitialCurrent=0  Capacitance=1e-6  Setx0=off  InitialVoltage=0  Measurements=None
  RnA2 : spsSeriesRLCBranchLib/Series RLC Branch  LConnTagsString=__new0  RConnTagsString=__new0  BranchType=R  Resistance=160  Inductance=1e-3  SetiL0=off  InitialCurrent=0  Capacitance=1e-6  Setx0=off  InitialVoltage=0  Measurements=None
  RpA : spsSeriesRLCBranchLib/Series RLC Branch  LConnTagsString=__new0  RConnTagsString=__new0  BranchType=R  Resistance=150  Inductance=1e-3  SetiL0=off  InitialCurrent=0  Capacitance=1e-6  Setx0=off  InitialVoltage=0  Measurements=None
  RpA1 : spsSeriesRLCBranchLib/Series RLC Branch  LConnTagsString=__new0  RConnTagsString=__new0  BranchType=R  Resistance=150  Inductance=1e-3  SetiL0=off  InitialCurrent=0  Capacitance=1e-6  Setx0=off  InitialVoltage=0  Measurements=None
  RpA2 : spsSeriesRLCBranchLib/Series RLC Branch  LConnTagsString=__new0  RConnTagsString=__new0  BranchType=R  Resistance=150  Inductance=1e-3  SetiL0=off  InitialCurrent=0  Capacitance=1e-6  Setx0=off  InitialVoltage=0  Measurements=None
  VnA : spsDCVoltageSourceLib/DC Voltage Source  Amplitude=2050  Measurements=None
  VnA1 : spsDCVoltageSourceLib/DC Voltage Source  Amplitude=2050  Measurements=None
  VnA2 : spsDCVoltageSourceLib/DC Voltage Source  Amplitude=2050  Measurements=None
  VpA : spsDCVoltageSourceLib/DC Voltage Source  Amplitude=2000  Measurements=None
  VpA1 : spsDCVoltageSourceLib/DC Voltage Source  Amplitude=2000  Measurements=None
  VpA2 : spsDCVoltageSourceLib/DC Voltage Source  Amplitude=2000  Measurements=None
  1 : PMIOPort  Side=Left
  2 : PMIOPort  Port=2  Side=Left
  3 : PMIOPort  Port=3  Side=Left
  connections:
  GndHIF3/LConn1 -- VpA1/LConn1
  DnA1/RConn1 -- DpA1/LConn1 -- BrkB/RConn1
  GndHIF5/LConn1 -- VpA2/LConn1
  VpA/RConn1 -- RpA/RConn1
  BrkA/LConn1 -- 1/RConn1
  DnA/LConn1 -- RnA/LConn1
  RnA1/RConn1 -- VnA1/LConn1
  DnA2/RConn1 -- DpA2/LConn1 -- BrkC/RConn1
  RnA2/RConn1 -- VnA2/LConn1
  VpA1/RConn1 -- RpA1/RConn1
  GndHIF2/LConn1 -- VnA1/RConn1
  DnA1/LConn1 -- RnA1/LConn1
  DpA2/RConn1 -- RpA2/LConn1
  GndHIF4/LConn1 -- VnA2/RConn1
  RnA/RConn1 -- VnA/LConn1
  VpA2/RConn1 -- RpA2/RConn1
  DnA2/LConn1 -- RnA2/LConn1
  DpA1/RConn1 -- RpA1/LConn1
  BrkA/RConn1 -- DpA/LConn1 -- DnA/RConn1
  GndHIF1/LConn1 -- VpA/LConn1
  DpA/RConn1 -- RpA/LConn1
  GndHIF/LConn1 -- VnA/RConn1
  2/RConn1 -- BrkB/LConn1
  3/RConn1 -- BrkC/LConn1

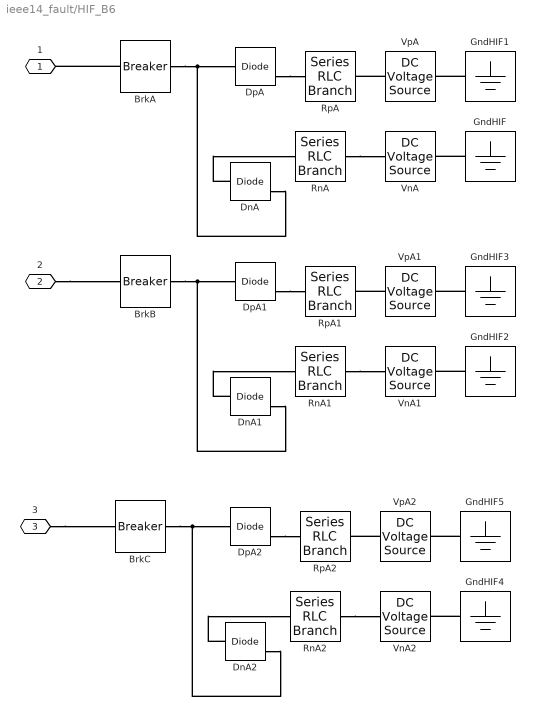
== system ieee14_fault/HIF_B6 ==
  BrkA : spsBreakerLib/Breaker  InitialState=0  SwitchingTimes=[100]  External=off  BreakerResistance=0.01  SnubberResistance=1e6  SnubberCapacitance=inf  Measurements=None  MoreParameters=on  NoBreakLoop=off
  BrkB : spsBreakerLib/Breaker  InitialState=0  SwitchingTimes=[100]  External=off  BreakerResistance=0.01  SnubberResistance=1e6  SnubberCapacitance=inf  Measurements=None  MoreParameters=on  NoBreakLoop=off
  BrkC : spsBreakerLib/Breaker  InitialState=0  SwitchingTimes=[100]  External=off  BreakerResistance=0.01  SnubberResistance=1e6  SnubberCapacitance=inf  Measurements=None  MoreParameters=on  NoBreakLoop=off
  DnA : spsDiodeLib/Diode  Ron=0.001  Lon=0  Vf=0.8  IC=0  UseSnubber=0  Rs=1e6  Cs=inf  Measurements=on
  DnA1 : spsDiodeLib/Diode  Ron=0.001  Lon=0  Vf=0.8  IC=0  UseSnubber=0  Rs=1e6  Cs=inf  Measurements=on
  DnA2 : spsDiodeLib/Diode  Ron=0.001  Lon=0  Vf=0.8  IC=0  UseSnubber=0  Rs=1e6  Cs=inf  Measurements=on
  DpA : spsDiodeLib/Diode  Ron=0.001  Lon=0  Vf=0.8  IC=0  UseSnubber=0  Rs=1e6  Cs=inf  Measurements=on
  DpA1 : spsDiodeLib/Diode  Ron=0.001  Lon=0  Vf=0.8  IC=0  UseSnubber=0  Rs=1e6  Cs=inf  Measurements=on
  DpA2 : spsDiodeLib/Diode  Ron=0.001  Lon=0  Vf=0.8  IC=0  UseSnubber=0  Rs=1e6  Cs=inf  Measurements=on
  GndHIF{,1..5} (6 alike) : spsGroundLib/Ground  LConnTagsString=a
  RnA : spsSeriesRLCBranchLib/Series RLC Branch  LConnTagsString=__new0  RConnTagsString=__new0  BranchType=R  Resistance=160  Inductance=1e-3  SetiL0=off  InitialCurrent=0  Capacitance=1e-6  Setx0=off  InitialVoltage=0  Measurements=None
  RnA1 : spsSeriesRLCBranchLib/Series RLC Branch  LConnTagsString=__new0  RConnTagsString=__new0  BranchType=R  Resistance=160  Inductance=1e-3  SetiL0=off  InitialCurrent=0  Capacitance=1e-6  Setx0=off  InitialVoltage=0  Measurements=None
  RnA2 : spsSeriesRLCBranchLib/Series RLC Branch  LConnTagsString=__new0  RConnTagsString=__new0  BranchType=R  Resistance=160  Inductance=1e-3  SetiL0=off  InitialCurrent=0  Capacitance=1e-6  Setx0=off  InitialVoltage=0  Measurements=None
  RpA : spsSeriesRLCBranchLib/Series RLC Branch  LConnTagsString=__new0  RConnTagsString=__new0  BranchType=R  Resistance=150  Inductance=1e-3  SetiL0=off  InitialCurrent=0  Capacitance=1e-6  Setx0=off  InitialVoltage=0  Measurements=None
  RpA1 : spsSeriesRLCBranchLib/Series RLC Branch  LConnTagsString=__new0  RConnTagsString=__new0  BranchType=R  Resistance=150  Inductance=1e-3  SetiL0=off  InitialCurrent=0  Capacitance=1e-6  Setx0=off  InitialVoltage=0  Measurements=None
  RpA2 : spsSeriesRLCBranchLib/Series RLC Branch  LConnTagsString=__new0  RConnTagsString=__new0  BranchType=R  Resistance=150  Inductance=1e-3  SetiL0=off  InitialCurrent=0  Capacitance=1e-6  Setx0=off  InitialVoltage=0  Measurements=None
  VnA : spsDCVoltageSourceLib/DC Voltage Source  Amplitude=2050  Measurements=None
  VnA1 : spsDCVoltageSourceLib/DC Voltage Source  Amplitude=2050  Measurements=None
  VnA2 : spsDCVoltageSourceLib/DC Voltage Source  Amplitude=2050  Measurements=None
  VpA : spsDCVoltageSourceLib/DC Voltage Source  Amplitude=2000  Measurements=None
  VpA1 : spsDCVoltageSourceLib/DC Voltage Source  Amplitude=2000  Measurements=None
  VpA2 : spsDCVoltageSourceLib/DC Voltage Source  Amplitude=2000  Measurements=None
  1 : PMIOPort  Side=Left
  2 : PMIOPort  Port=2  Side=Left
  3 : PMIOPort  Port=3  Side=Left
  connections:
  GndHIF3/LConn1 -- VpA1/LConn1
  DnA1/RConn1 -- DpA1/LConn1 -- BrkB/RConn1
  GndHIF5/LConn1 -- VpA2/LConn1
  VpA/RConn1 -- RpA/RConn1
  BrkA/LConn1 -- 1/RConn1
  DnA/LConn1 -- RnA/LConn1
  RnA1/RConn1 -- VnA1/LConn1
  DnA2/RConn1 -- DpA2/LConn1 -- BrkC/RConn1
  RnA2/RConn1 -- VnA2/LConn1
  VpA1/RConn1 -- RpA1/RConn1
  GndHIF2/LConn1 -- VnA1/RConn1
  DnA1/LConn1 -- RnA1/LConn1
  DpA2/RConn1 -- RpA2/LConn1
  GndHIF4/LConn1 -- VnA2/RConn1
  RnA/RConn1 -- VnA/LConn1
  VpA2/RConn1 -- RpA2/RConn1
  DnA2/LConn1 -- RnA2/LConn1
  DpA1/RConn1 -- RpA1/LConn1
  BrkA/RConn1 -- DpA/LConn1 -- DnA/RConn1
  GndHIF1/LConn1 -- VpA/LConn1
  DpA/RConn1 -- RpA/LConn1
  GndHIF/LConn1 -- VnA/RConn1
  2/RConn1 -- BrkB/LConn1
  3/RConn1 -- BrkC/LConn1

== system ieee14_fault/HIF_B7 ==
  BrkA : spsBreakerLib/Breaker  InitialState=0  SwitchingTimes=[100]  External=off  BreakerResistance=0.01  SnubberResistance=1e6  SnubberCapacitance=inf  Measurements=None  MoreParameters=on  NoBreakLoop=off
  BrkB : spsBreakerLib/Breaker  InitialState=0  SwitchingTimes=[100]  External=off  BreakerResistance=0.01  SnubberResistance=1e6  SnubberCapacitance=inf  Measurements=None  MoreParameters=on  NoBreakLoop=off
  BrkC : spsBreakerLib/Breaker  InitialState=0  SwitchingTimes=[100]  External=off  BreakerResistance=0.01  SnubberResistance=1e6  SnubberCapacitance=inf  Measurements=None  MoreParameters=on  NoBreakLoop=off
  DnA : spsDiodeLib/Diode  Ron=0.001  Lon=0  Vf=0.8  IC=0  UseSnubber=0  Rs=1e6  Cs=inf  Measurements=on
  DnA1 : spsDiodeLib/Diode  Ron=0.001  Lon=0  Vf=0.8  IC=0  UseSnubber=0  Rs=1e6  Cs=inf  Measurements=on
  DnA2 : spsDiodeLib/Diode  Ron=0.001  Lon=0  Vf=0.8  IC=0  UseSnubber=0  Rs=1e6  Cs=inf  Measurements=on
  DpA : spsDiodeLib/Diode  Ron=0.001  Lon=0  Vf=0.8  IC=0  UseSnubber=0  Rs=1e6  Cs=inf  Measurements=on
  DpA1 : spsDiodeLib/Diode  Ron=0.001  Lon=0  Vf=0.8  IC=0  UseSnubber=0  Rs=1e6  Cs=inf  Measurements=on
  DpA2 : spsDiodeLib/Diode  Ron=0.001  Lon=0  Vf=0.8  IC=0  UseSnubber=0  Rs=1e6  Cs=inf  Measurements=on
  GndHIF{,1..5} (6 alike) : spsGroundLib/Ground  LConnTagsString=a
  RnA : spsSeriesRLCBranchLib/Series RLC Branch  LConnTagsString=__new0  RConnTagsString=__new0  BranchType=R  Resistance=160  Inductance=1e-3  SetiL0=off  InitialCurrent=0  Capacitance=1e-6  Setx0=off  InitialVoltage=0  Measurements=None
  RnA1 : spsSeriesRLCBranchLib/Series RLC Branch  LConnTagsString=__new0  RConnTagsString=__new0  BranchType=R  Resistance=160  Inductance=1e-3  SetiL0=off  InitialCurrent=0  Capacitance=1e-6  Setx0=off  InitialVoltage=0  Measurements=None
  RnA2 : spsSeriesRLCBranchLib/Series RLC Branch  LConnTagsString=__new0  RConnTagsString=__new0  BranchType=R  Resistance=160  Inductance=1e-3  SetiL0=off  InitialCurrent=0  Capacitance=1e-6  Setx0=off  InitialVoltage=0  Measurements=None
  RpA : spsSeriesRLCBranchLib/Series RLC Branch  LConnTagsString=__new0  RConnTagsString=__new0  BranchType=R  Resistance=150  Inductance=1e-3  SetiL0=off  InitialCurrent=0  Capacitance=1e-6  Setx0=off  InitialVoltage=0  Measurements=None
  RpA1 : spsSeriesRLCBranchLib/Series RLC Branch  LConnTagsString=__new0  RConnTagsString=__new0  BranchType=R  Resistance=150  Inductance=1e-3  SetiL0=off  InitialCurrent=0  Capacitance=1e-6  Setx0=off  InitialVoltage=0  Measurements=None
  RpA2 : spsSeriesRLCBranchLib/Series RLC Branch  LConnTagsString=__new0  RConnTagsString=__new0  BranchType=R  Resistance=150  Inductance=1e-3  SetiL0=off  InitialCurrent=0  Capacitance=1e-6  Setx0=off  InitialVoltage=0  Measurements=None
  VnA : spsDCVoltageSourceLib/DC Voltage Source  Amplitude=2050  Measurements=None
  VnA1 : spsDCVoltageSourceLib/DC Voltage Source  Amplitude=2050  Measurements=None
  VnA2 : spsDCVoltageSourceLib/DC Voltage Source  Amplitude=2050  Measurements=None
  VpA : spsDCVoltageSourceLib/DC Voltage Source  Amplitude=2000  Measurements=None
  VpA1 : spsDCVoltageSourceLib/DC Voltage Source  Amplitude=2000  Measurements=None
  VpA2 : spsDCVoltageSourceLib/DC Voltage Source  Amplitude=2000  Measurements=None
  1 : PMIOPort  Side=Left
  2 : PMIOPort  Port=2  Side=Left
  3 : PMIOPort  Port=3  Side=Left
  connections:
  GndHIF3/LConn1 -- VpA1/LConn1
  DnA1/RConn1 -- DpA1/LConn1 -- BrkB/RConn1
  GndHIF5/LConn1 -- VpA2/LConn1
  VpA/RConn1 -- RpA/RConn1
  BrkA/LConn1 -- 1/RConn1
  DnA/LConn1 -- RnA/LConn1
  RnA1/RConn1 -- VnA1/LConn1
  DnA2/RConn1 -- DpA2/LConn1 -- BrkC/RConn1
  RnA2/RConn1 -- VnA2/LConn1
  VpA1/RConn1 -- RpA1/RConn1
  GndHIF2/LConn1 -- VnA1/RConn1
  DnA1/LConn1 -- RnA1/LConn1
  DpA2/RConn1 -- RpA2/LConn1
  GndHIF4/LConn1 -- VnA2/RConn1
  RnA/RConn1 -- VnA/LConn1
  VpA2/RConn1 -- RpA2/RConn1
  DnA2/LConn1 -- RnA2/LConn1
  DpA1/RConn1 -- RpA1/LConn1
  BrkA/RConn1 -- DpA/LConn1 -- DnA/RConn1
  GndHIF1/LConn1 -- VpA/LConn1
  DpA/RConn1 -- RpA/LConn1
  GndHIF/LConn1 -- VnA/RConn1
  2/RConn1 -- BrkB/LConn1
  3/RConn1 -- BrkC/LConn1

== system ieee14_fault/HIF_B8 ==
  BrkA : spsBreakerLib/Breaker  InitialState=0  SwitchingTimes=[100]  External=off  BreakerResistance=0.01  SnubberResistance=1e6  SnubberCapacitance=inf  Measurements=None  MoreParameters=on  NoBreakLoop=off
  BrkB : spsBreakerLib/Breaker  InitialState=0  SwitchingTimes=[100]  External=off  BreakerResistance=0.01  SnubberResistance=1e6  SnubberCapacitance=inf  Measurements=None  MoreParameters=on  NoBreakLoop=off
  BrkC : spsBreakerLib/Breaker  InitialState=0  SwitchingTimes=[100]  External=off  BreakerResistance=0.01  SnubberResistance=1e6  SnubberCapacitance=inf  Measurements=None  MoreParameters=on  NoBreakLoop=off
  DnA : spsDiodeLib/Diode  Ron=0.001  Lon=0  Vf=0.8  IC=0  UseSnubber=0  Rs=1e6  Cs=inf  Measurements=on
  DnA1 : spsDiodeLib/Diode  Ron=0.001  Lon=0  Vf=0.8  IC=0  UseSnubber=0  Rs=1e6  Cs=inf  Measurements=on
  DnA2 : spsDiodeLib/Diode  Ron=0.001  Lon=0  Vf=0.8  IC=0  UseSnubber=0  Rs=1e6  Cs=inf  Measurements=on
  DpA : spsDiodeLib/Diode  Ron=0.001  Lon=0  Vf=0.8  IC=0  UseSnubber=0  Rs=1e6  Cs=inf  Measurements=on
  DpA1 : spsDiodeLib/Diode  Ron=0.001  Lon=0  Vf=0.8  IC=0  UseSnubber=0  Rs=1e6  Cs=inf  Measurements=on
  DpA2 : spsDiodeLib/Diode  Ron=0.001  Lon=0  Vf=0.8  IC=0  UseSnubber=0  Rs=1e6  Cs=inf  Measurements=on
  GndHIF{,1..5} (6 alike) : spsGroundLib/Ground  LConnTagsString=a
  RnA : spsSeriesRLCBranchLib/Series RLC Branch  LConnTagsString=__new0  RConnTagsString=__new0  BranchType=R  Resistance=160  Inductance=1e-3  SetiL0=off  InitialCurrent=0  Capacitance=1e-6  Setx0=off  InitialVoltage=0  Measurements=None
  RnA1 : spsSeriesRLCBranchLib/Series RLC Branch  LConnTagsString=__new0  RConnTagsString=__new0  BranchType=R  Resistance=160  Inductance=1e-3  SetiL0=off  InitialCurrent=0  Capacitance=1e-6  Setx0=off  InitialVoltage=0  Measurements=None
  RnA2 : spsSeriesRLCBranchLib/Series RLC Branch  LConnTagsString=__new0  RConnTagsString=__new0  BranchType=R  Resistance=160  Inductance=1e-3  SetiL0=off  InitialCurrent=0  Capacitance=1e-6  Setx0=off  InitialVoltage=0  Measurements=None
  RpA : spsSeriesRLCBranchLib/Series RLC Branch  LConnTagsString=__new0  RConnTagsString=__new0  BranchType=R  Resistance=150  Inductance=1e-3  SetiL0=off  InitialCurrent=0  Capacitance=1e-6  Setx0=off  InitialVoltage=0  Measurements=None
  RpA1 : spsSeriesRLCBranchLib/Series RLC Branch  LConnTagsString=__new0  RConnTagsString=__new0  BranchType=R  Resistance=150  Inductance=1e-3  SetiL0=off  InitialCurrent=0  Capacitance=1e-6  Setx0=off  InitialVoltage=0  Measurements=None
  RpA2 : spsSeriesRLCBranchLib/Series RLC Branch  LConnTagsString=__new0  RConnTagsString=__new0  BranchType=R  Resistance=150  Inductance=1e-3  SetiL0=off  InitialCurrent=0  Capacitance=1e-6  Setx0=off  InitialVoltage=0  Measurements=None
  VnA : spsDCVoltageSourceLib/DC Voltage Source  Amplitude=2050  Measurements=None
  VnA1 : spsDCVoltageSourceLib/DC Voltage Source  Amplitude=2050  Measurements=None
  VnA2 : spsDCVoltageSourceLib/DC Voltage Source  Amplitude=2050  Measurements=None
  VpA : spsDCVoltageSourceLib/DC Voltage Source  Amplitude=2000  Measurements=None
  VpA1 : spsDCVoltageSourceLib/DC Voltage Source  Amplitude=2000  Measurements=None
  VpA2 : spsDCVoltageSourceLib/DC Voltage Source  Amplitude=2000  Measurements=None
  1 : PMIOPort  Side=Left
  2 : PMIOPort  Port=2  Side=Left
  3 : PMIOPort  Port=3  Side=Left
  connections:
  GndHIF3/LConn1 -- VpA1/LConn1
  DnA1/RConn1 -- DpA1/LConn1 -- BrkB/RConn1
  GndHIF5/LConn1 -- VpA2/LConn1
  VpA/RConn1 -- RpA/RConn1
  BrkA/LConn1 -- 1/RConn1
  DnA/LConn1 -- RnA/LConn1
  RnA1/RConn1 -- VnA1/LConn1
  DnA2/RConn1 -- DpA2/LConn1 -- BrkC/RConn1
  RnA2/RConn1 -- VnA2/LConn1
  VpA1/RConn1 -- RpA1/RConn1
  GndHIF2/LConn1 -- VnA1/RConn1
  DnA1/LConn1 -- RnA1/LConn1
  DpA2/RConn1 -- RpA2/LConn1
  GndHIF4/LConn1 -- VnA2/RConn1
  RnA/RConn1 -- VnA/LConn1
  VpA2/RConn1 -- RpA2/RConn1
  DnA2/LConn1 -- RnA2/LConn1
  DpA1/RConn1 -- RpA1/LConn1
  BrkA/RConn1 -- DpA/LConn1 -- DnA/RConn1
  GndHIF1/LConn1 -- VpA/LConn1
  DpA/RConn1 -- RpA/LConn1
  GndHIF/LConn1 -- VnA/RConn1
  2/RConn1 -- BrkB/LConn1
  3/RConn1 -- BrkC/LConn1
